simulink model "EVIDS_core"  (R2021b)
settings: Solver=FixedStepAuto  StartTime=0.0  StopTime=5  FixedStep=0.001  RelTol=1e-3
PreLoadFcn:
  | evids_test_initialize('EVIDS_core','load');
PostLoadFcn:
  | addpath(fileparts(get_param('EVIDS_core','FileName')));
InitFcn:
  | evids_test_initialize('EVIDS_core');
StopFcn:
  | evids_test_schedule_results('EVIDS_core');
libraries: Solver_SF x1
settings Model: Creator=15337  LastModifiedBy=15337
settings DataIOCC: SaveOutput=off  ReturnWorkspaceOutputs=off  TimeSaveName=evids_time  SignalLoggingName=evids_logsout

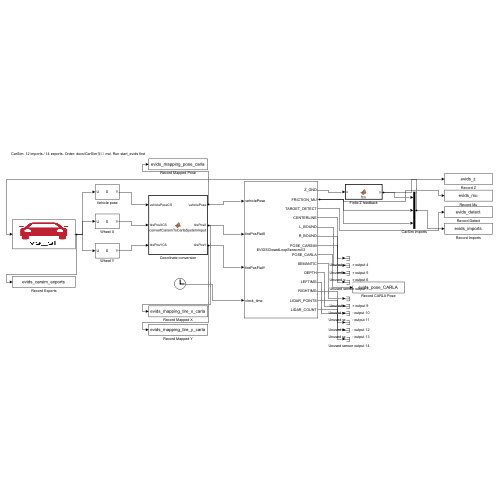
[thumbnail: Simulink's stored preview of the top-level diagram]
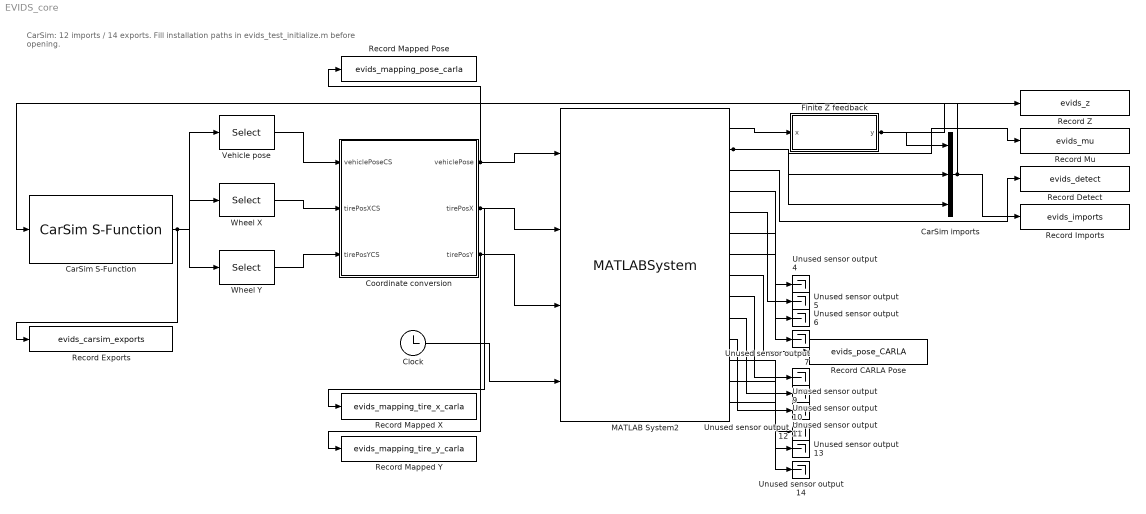
== system EVIDS_core ==
  note: CarSim: 12 imports / 14 exports. Fill installation paths in evids_test_initialize.m before opening.
  CarSim S-Function : Solver_SF/CarSim S-Function  Priority=1  SIMFILE=simfile.sim  Run_RTs=off  vs_state_ind=Run  StopMode_ind=Vehicle Model
  CarSim imports : Mux  Inputs=3
  Clock : Clock
  Coordinate conversion : MATLAB Function  TreatAsAtomicUnit=on
  Finite Z feedback : MATLAB Function  TreatAsAtomicUnit=on
  MATLAB System2 : MATLABSystem  System=EVIDSClosedLoopSensorsV2  SpawnX=0  SpawnY=0  SpawnZ=0.0  SimulinkDt=0.001  RaycastDt=0.01  FarRaycastDt=0.1  RayNearMargin=3  RayExitHysteresis=2  RayApproachSpeed=80  CarlaDt=0.05  RoadFriction=1.0  FilterAlpha=1  EnableSave=false  SavePeriod=0.05  CameraHeight=1.2  CameraX=1.5  CameraYOffset=0.5  CameraFOV=90  LaneSamplePoints=50  LaneSampleDist=2.0  ViewMode=1  CarlaHost=localhost  CarlaPort=2000  PropConfigurationFunction=evids_test_props  EnableSemantic=false  EnableDepth=false  EnableStereoRGB=false  EnableLidar=false  LidarMaxPoints=30000  SimulateUsing=Interpreted execution
      mask Type: EVIDSClosedLoopSensorsV2
      mask Display:
      | disp('EVIDSClosedLoopSensorsV2');
      | port_label('input',1,'vehiclePose');
      | port_label('input',2,'tirePosFlatX');
      | port_label('input',3,'tirePosFlatY');
      | port_label('input',4,'clock_time');
      | port_label('output',1,'Z_GND');
      | port_label('output',2,'FRICTION_MU');
      | port_label('output',3,'TARGET_DETECT');
      | port_label('output',4,'CENTERLINE');
      | port_label('output',5,'L_BOUND');
      | port_label('output',6,'R_BOUND');
      | port_label('output',7,'POSE_CARSIM');
      | port_label('output',8,'POSE_CARLA');
      | port_label('output',9,'SEMANTIC');
      | port_label('output',10,'DEPTH');
      | port_label('output',11,'LEFTIMG');
      | port_label('output',12,'RIGHTIMG');
      | port_label('output',13,'LIDAR_POINTS');
      | port_label('output',14,'LIDAR_COUNT');
  Record CARLA Pose : ToWorkspace  VariableName=evids_pose_CARLA  SaveFormat=Timeseries  SampleTime=-1
  Record Detect : ToWorkspace  VariableName=evids_detect  SaveFormat=Timeseries  SampleTime=-1
  Record Exports : ToWorkspace  VariableName=evids_carsim_exports  SaveFormat=Timeseries  SampleTime=-1
  Record Imports : ToWorkspace  VariableName=evids_imports  SaveFormat=Timeseries  SampleTime=-1
  Record Mapped Pose : ToWorkspace  VariableName=evids_mapping_pose_carla  SaveFormat=Timeseries  SampleTime=-1
  Record Mapped X : ToWorkspace  VariableName=evids_mapping_tire_x_carla  SaveFormat=Timeseries  SampleTime=-1
  Record Mapped Y : ToWorkspace  VariableName=evids_mapping_tire_y_carla  SaveFormat=Timeseries  SampleTime=-1
  Record Mu : ToWorkspace  VariableName=evids_mu  SaveFormat=Timeseries  SampleTime=-1
  Record Z : ToWorkspace  VariableName=evids_z  SaveFormat=Timeseries  SampleTime=-1
  Unused sensor output {4..7,9..14} (10 alike) : Terminator
  Vehicle pose : Selector  InputPortWidth=14  IndexOptions=Index vector (dialog)  Indices=[1 2 3 4 5 6]  OutputSizes=1
  Wheel X : Selector  InputPortWidth=14  IndexOptions=Index vector (dialog)  Indices=[7 9 11 13]  OutputSizes=1
  Wheel Y : Selector  InputPortWidth=14  IndexOptions=Index vector (dialog)  Indices=[8 10 12 14]  OutputSizes=1
  wires:
  CarSim S-Function/1 -> Vehicle pose/1, Wheel X/1, Wheel Y/1, Record Exports/1
  Vehicle pose/1 -> Coordinate conversion/1(vehiclePoseCS)
  Wheel X/1 -> Coordinate conversion/2(tirePosXCS)
  Wheel Y/1 -> Coordinate conversion/3(tirePosYCS)
  Coordinate conversion/1(vehiclePose) -> MATLAB System2/1, Record Mapped Pose/1
  Coordinate conversion/2(tirePosX) -> MATLAB System2/2, Record Mapped X/1
  Coordinate conversion/3(tirePosY) -> MATLAB System2/3, Record Mapped Y/1
  Clock/1 -> MATLAB System2/4
  MATLAB System2/1 -> Finite Z feedback/1(x)
  Finite Z feedback/1(y) -> CarSim imports/1, Record Z/1
  MATLAB System2/2 -> CarSim imports/2, CarSim imports/3, Record Mu/1
  CarSim imports/1 -> CarSim S-Function/1, Record Imports/1
  MATLAB System2/3 -> Record Detect/1
  MATLAB System2/8 -> Record CARLA Pose/1
  MATLAB System2/4 -> Unused sensor output 4/1
  MATLAB System2/5 -> Unused sensor output 5/1
  MATLAB System2/6 -> Unused sensor output 6/1
  MATLAB System2/7 -> Unused sensor output 7/1
  MATLAB System2/9 -> Unused sensor output 9/1
  MATLAB System2/10 -> Unused sensor output 10/1
  MATLAB System2/11 -> Unused sensor output 11/1
  MATLAB System2/12 -> Unused sensor output 12/1
  MATLAB System2/13 -> Unused sensor output 13/1
  MATLAB System2/14 -> Unused sensor output 14/1

== matlab function EVIDS_core/Coordinate conversion ==
  data: vehiclePoseCS input; vehiclePose output; tirePosXCS input; tirePosYCS input; tirePosX output; tirePosY output
function [vehiclePose, tirePosX, tirePosY] = convertCarsimToCarlaSystemInput(vehiclePoseCS, tirePosXCS, tirePosYCS)
% Code generation compatible version.
% Inputs:
%   vehiclePoseCS : 6x1 or 1x6, [X,Y,Z,Pitch,Roll,Yaw]
%   tirePosXCS    : 4x1 or 1x4, [L1,R1,L2,R2]
%   tirePosYCS    : 4x1 or 1x4, [L1,R1,L2,R2]
%
% Outputs:
%   vehiclePose   : 6x1, converted [X,Y,Z,Pitch,Roll,Yaw]
%   tirePosX      : 4x1, converted [L1,R1,L2,R2]
%   tirePosY      : 4x1, converted [L1,R1,L2,R2]

% ============================================================
% Configuration

% CarSim and CARLA have opposite lateral semantics, so mirror laterally.
mirrorSign = -1.0;

% ============================================================
% Persistent reference values from the first frame
% ============================================================
persistent refX0 refY0 yawRef0 isInitialized

if isempty(isInitialized)
    isInitialized = false;
    refX0 = 0.0;
    refY0 = 0.0;
    yawRef0 = 0.0;
end

% ============================================================
% Fixed-size output initialization
% ============================================================
vehiclePose = zeros(6,1);
tirePosX    = zeros(4,1);
tirePosY    = zeros(4,1);

% ============================================================
% Convert inputs to column vectors
% ============================================================
vehiclePoseCS_col = vehiclePoseCS(:);
tirePosXCS_col    = tirePosXCS(:);
tirePosYCS_col    = tirePosYCS(:);

% ============================================================
% First-frame initialization
% ============================================================
if ~isInitialized
    refX0   = double(vehiclePoseCS_col(1));
    refY0   = double(vehiclePoseCS_col(2));
    yawRef0 = double(vehiclePoseCS_col(6));
    isInitialized = true;
end

% ============================================================
% Current frame vehicle pose from CarSim
% ============================================================
xCS     = double(vehiclePoseCS_col(1));
yCS     = double(vehiclePoseCS_col(2));
zCS     = double(vehiclePoseCS_col(3));
pitchCS = double(vehiclePoseCS_col(4));
rollCS  = double(vehiclePoseCS_col(5));
yawCS   = double(vehiclePoseCS_col(6));

% ============================================================
% Reference basis from first-frame yaw
% ============================================================
fRefX = cosd(yawRef0);
fRefY = sind(yawRef0);

normF = sqrt(fRefX*fRefX + fRefY*fRefY);
fRefX = fRefX / normF;
fRefY = fRefY / normF;

% CARLA left direction:
% forward = [cos(yaw), sin(yaw)]
% right   = [-sin(yaw), cos(yaw)]
% left    = [sin(yaw), -cos(yaw)]
leftRefX = sind(yawRef0);
leftRefY = -cosd(yawRef0);

normL = sqrt(leftRefX*leftRefX + leftRefY*leftRefY);
leftRefX = leftRefX / normL;
leftRefY = leftRefY / normL;

% ============================================================
% Transform vehicle center position
% ============================================================
[xCarla, yCarla] = transformPointByLateralMirrorScalar( ...
    xCS, yCS, refX0, refY0, fRefX, fRefY, leftRefX, leftRefY, mirrorSign);

zCarla = zCS;

% ============================================================
% Transform four tire positions
% ============================================================
for i = 1:4
    [tx, ty] = transformPointByLateralMirrorScalar( ...
        double(tirePosXCS_col(i)), ...
        double(tirePosYCS_col(i)), ...
        refX0, refY0, ...
        fRefX, fRefY, ...
        leftRefX, leftRefY, ...
        mirrorSign);

    tirePosX(i) = tx;
    tirePosY(i) = ty;
end

% ============================================================
% Transform attitude angles
% ============================================================
yawCarla = wrapTo180Local(2.0 * yawRef0 - yawCS);

% Pitch remains physically unchanged.
pitchCarla = -pitchCS;

% Roll changes sign because the lateral direction is mirrored.
rollCarla = rollCS;

% ============================================================
% Output vehiclePose
% ============================================================
vehiclePose(1) = xCarla;
vehiclePose(2) = yCarla;
vehiclePose(3) = zCarla;
vehiclePose(4) = pitchCarla;
vehiclePose(5) = rollCarla;
vehiclePose(6) = yawCarla;

end

% ========================================================================
% Local functions
% ========================================================================

function [xOut, yOut] = transformPointByLateralMirrorScalar( ...
    xIn, yIn, refX, refY, fRefX, fRefY, leftRefX, leftRefY, mirrorSign)
% Mirror a point about the reference axis.
%
% rel = p - p0
% s   = dot(rel, fRef)
% d   = dot(rel, leftRef)
% relOut = s*fRef + mirrorSign*d*leftRef
%
% mirrorSign = -1 means lateral mirror.

relX = xIn - refX;
relY = yIn - refY;

s = relX * fRefX + relY * fRefY;
d = relX * leftRefX + relY * leftRefY;

relOutX = s * fRefX + mirrorSign * d * leftRefX;
relOutY = s * fRefY + mirrorSign * d * leftRefY;

xOut = refX + relOutX;
yOut = refY + relOutY;

end

function ang = wrapTo180Local(ang)
% Wrap angle to [-180, 180).

ang = mod(ang + 180.0, 360.0) - 180.0;

end

== matlab function EVIDS_core/Finite Z feedback ==
  data: x input; y output
function y = fcn(x)
    % 找到 x 中所有为 NaN 的位置，并将其赋值为 0
    x(isnan(x)) = 0;
    
    % 将处理后的矩阵赋值给输出变量 y
    y = x;
end
